simulink model "arducopter"  (R2024b)
settings: Solver=FixedStepAuto  StartTime=0.0  StopTime=simIn.param.timeEnd  FixedStep=simIn.param.dt  RelTol=1e-3
undefined symbols (not defined in the file or in its folder): DiscIntNeverNeededParam, sim, simIn
libraries: simulink x60, slident x4, vrlib x1
(part 6 of 9)

== system arducopter/Rate Controller/PID Yaw Rate/Slew Limiter ==
  note: Data Store Memory Elements: Global variables of subsystem
  note: Slew Limiter
      |
      | Calculates the slew limit modifiert Dmod for the P and D part of the controller. The calculation of Dmod is taken from SlewLimiter::modifier() in SlewLimiter.cpp.
  note: Alpha Calculation:
      | $\alpha = \frac{\mathrm{d}t}{\mathrm{d}t + 2 \pi f_{\mathrm{Cutoff}}$
  note: See AP_Math.cpp, calc_lowpass_alpha_dt()
  p_out : Inport
  sr_max : Inport  Port=2
  sr_tau : Inport  Port=3
  sr_flt_f : Inport  Port=4
  clock : Inport  Port=5
  d_out : Inport  Port=6
  ATC input time constant : Constant  Value=simIn.param.dt
  Add1 : Sum
  Calculate Alpha : Product  Inputs=*/
  Calculate Dmod : MATLAB Function  TreatAsAtomicUnit=on  SystemSampleTime=0.0025
  Compare To Zero2 : simulink/Logic and Bit Operations/Compare To Zero  relop=<=  OutDataTypeStr=boolean
  Compare To Zero3 : simulink/Logic and Bit Operations/Compare To Zero  relop=<=  OutDataTypeStr=boolean
  Compare To Zero4 : simulink/Logic and Bit Operations/Compare To Zero  relop=~=  OutDataTypeStr=boolean
  Constant1 : Constant  OutDataTypeStr=single
  Constant5 : Constant  OutDataTypeStr=single
  Data Store Memory : DataStoreMemory  DataStoreName=pos_event_stored  ReadBeforeWriteMsg=warning  WriteAfterWriteMsg=warning  WriteAfterReadMsg=warning  InitialValue=false  ShowAdditionalParam=off  OutDataTypeStr=boolean
  Data Store Memory1 : DataStoreMemory  DataStoreName=neg_event_stored  ReadBeforeWriteMsg=warning  WriteAfterWriteMsg=warning  WriteAfterReadMsg=warning  InitialValue=false  ShowAdditionalParam=off  OutDataTypeStr=boolean
  Data Store Memory10 : DataStoreMemory  DataStoreName=modifier_slew_rate  ReadBeforeWriteMsg=warning  WriteAfterWriteMsg=warning  WriteAfterReadMsg=warning  InitialValue=simIn.init.PIDY.SROut  ShowAdditionalParam=off  OutDataTypeStr=single
  Data Store Memory11 : DataStoreMemory  DataStoreName=output_slew_rate  ReadBeforeWriteMsg=warning  WriteAfterWriteMsg=warning  WriteAfterReadMsg=warning  InitialValue=simIn.init.PIDY.SROut  ShowAdditionalParam=off  OutDataTypeStr=single
  Data Store Memory2 : DataStoreMemory  DataStoreName=pos_event_idx  ReadBeforeWriteMsg=warning  WriteAfterWriteMsg=warning  WriteAfterReadMsg=warning  InitialValue=1  ShowAdditionalParam=off  OutDataTypeStr=int8
  Data Store Memory3 : DataStoreMemory  DataStoreName=neg_event_idx  ReadBeforeWriteMsg=warning  WriteAfterWriteMsg=warning  WriteAfterReadMsg=warning  InitialValue=1  ShowAdditionalParam=off  OutDataTypeStr=int8
  Data Store Memory4 : DataStoreMemory  DataStoreName=pos_event_ms  ReadBeforeWriteMsg=warning  WriteAfterWriteMsg=warning  WriteAfterReadMsg=warning  InitialValue=[0 0]  ShowAdditionalParam=off  OutDataTypeStr=uint32  Dimensions=2
  Data Store Memory5 : DataStoreMemory  DataStoreName=neg_event_ms  ReadBeforeWriteMsg=warning  WriteAfterWriteMsg=warning  WriteAfterReadMsg=warning  InitialValue=[0 0]  ShowAdditionalParam=off  OutDataTypeStr=uint32  Dimensions=2
  Data Store Memory6 : DataStoreMemory  DataStoreName=max_pos_slew_rate  ReadBeforeWriteMsg=warning  WriteAfterWriteMsg=warning  WriteAfterReadMsg=warning  ShowAdditionalParam=off  OutDataTypeStr=single
  Data Store Memory7 : DataStoreMemory  DataStoreName=max_pos_slew_event_ms  ReadBeforeWriteMsg=warning  WriteAfterWriteMsg=warning  WriteAfterReadMsg=warning  ShowAdditionalParam=off  OutDataTypeStr=uint32
  Data Store Memory8 : DataStoreMemory  DataStoreName=max_neg_slew_rate  ReadBeforeWriteMsg=warning  WriteAfterWriteMsg=warning  WriteAfterReadMsg=warning  ShowAdditionalParam=off  OutDataTypeStr=single
  Data Store Memory9 : DataStoreMemory  DataStoreName=max_neg_slew_event_ms  ReadBeforeWriteMsg=warning  WriteAfterWriteMsg=warning  WriteAfterReadMsg=warning  ShowAdditionalParam=off  OutDataTypeStr=uint32
  Data Store Read : DataStoreRead  DataStoreName=modifier_slew_rate  DataStoreElements=modifier_slew_rate  IndexOptions=Index vector (dialog)  Indices=1  OutputSizes=1
  Data Store Read1 : DataStoreRead  DataStoreName=output_slew_rate  DataStoreElements=output_slew_rate  IndexOptions=Index vector (dialog)  Indices=1  OutputSizes=1
  Data Type Conversion2 : DataTypeConversion  OutDataTypeStr=single  SaturateOnIntegerOverflow=off  RndMeth=Floor
  Divide1 : Product  Inputs=*/
  Gain1 : Gain  Gain=2*pi
  IC : InitialCondition  Value=2*simIn.init.PIDY.SROut
  Logical Operator1 : Logic  Operator=OR  AllPortsSameDT=off  OutDataTypeStr=boolean
  Lowpass Filter : MATLAB Function  TreatAsAtomicUnit=on
  Product2 : Product
  Subsystem : Subsystem
  Switch1 : Switch  Criteria=u2 > Threshold  SaturateOnIntegerOverflow=off  InputSameDT=off
  Terminator : Terminator
  Terminator1 : Terminator
  Unit Delay1 : UnitDelay  SampleTime=-1  HasFrameUpgradeWarning=on
  Dmod : Outport
  wires:
  Lowpass Filter/1(out) -> IC/1  "yawRateSrFilt"
  Unit Delay1/1 -> Lowpass Filter/3(out_last)
  Calculate Dmod/1(Dmod) -> Dmod/1  "yawRateDmod"
  sr_max/1 -> Calculate Dmod/2(sr_max)
  sr_tau/1 -> Calculate Dmod/3(sr_tau)
  Data Store Read/1 -> Terminator/1  "yawRateSrModifier"
  Data Store Read1/1 -> Terminator1/1  "yawRateSrOut"
  p_out/1 -> Subsystem/1(p_out)
  d_out/1 -> Subsystem/2(d_out)
  Subsystem/1(sr_raw) -> Lowpass Filter/1(in)  "yawRateSrRaw"
  IC/1 -> Calculate Dmod/1(slew_rate), Unit Delay1/1
  clock/1 -> Calculate Dmod/5(time)
  [cutoff_freq] -> Gain1/1
  [dt] -> Calculate Alpha/1, Add1/1
  Calculate Alpha/1 -> Switch1/3
  Gain1/1 -> Divide1/2
  Data Type Conversion2/1 -> [dt]
  ATC input time constant/1 -> Data Type Conversion2/1
  [cutoff_freq] -> Compare To Zero3/1
  Compare To Zero3/1 -> Logical Operator1/2
  Constant1/1 -> Divide1/1
  [dt] -> Compare To Zero2/1
  Logical Operator1/1 -> Switch1/2
  Compare To Zero2/1 -> Logical Operator1/1
  Add1/1 -> Calculate Alpha/2
  Divide1/1 -> Add1/2
  Product2/1 -> Switch1/1
  [dt] -> Compare To Zero4/1
  Switch1/1 -> Lowpass Filter/2(alpha)
  Compare To Zero4/1 -> Product2/1
  Constant5/1 -> Product2/2
  sr_flt_f/1 -> [cutoff_freq]
  [dt] -> Calculate Dmod/4(dt)

== system arducopter/Throttle/Throttle Calculations/Air density Calculation ==
  note: Calculation of the air density from the barometer signals.
      |
      | In order to determine the compensation gain, the air density ratio is calculated in this subsystem from the barometer measurement signals. This subsystem is only used for validation purposes.
      |
      | The calculations are based on the get_air_density_ratio() function in AP_AHRS.cpp and the _get_EAS2TAS() function (AP_Baro_atmosphere.cpp), which is called from there. The variable air_density_ratio for the air density ratio, which is used for the calculation of the compensation gain, is set in the ahrs() object.
  baroAlt : Inport
  baroAirPress : Inport  Port=2
  baroGndTemp : Inport  Port=3
  Data Store Memory : DataStoreMemory  DataStoreName=EAS2TAS  ReadBeforeWriteMsg=warning  WriteAfterWriteMsg=warning  WriteAfterReadMsg=warning  ShowAdditionalParam=off  OutDataTypeStr=single
  Data Store Memory1 : DataStoreMemory  DataStoreName=last_alt_EAS2TAS  ReadBeforeWriteMsg=warning  WriteAfterWriteMsg=warning  WriteAfterReadMsg=warning  ShowAdditionalParam=off  OutDataTypeStr=single
  Get air density ratio : MATLAB Function  TreatAsAtomicUnit=on
  Get equivalent to true airspeed EAS2TAS : MATLAB Function  TreatAsAtomicUnit=on  SystemSampleTime=simIn.param.dt
  airDensityRatio : Outport
  wires:
  Get equivalent to true airspeed EAS2TAS/1(eas2tas) -> Get air density ratio/1(eas2tas)
  Get air density ratio/1(airDensityRatio) -> airDensityRatio/1
  baroAlt/1 -> Get equivalent to true airspeed EAS2TAS/1(alt)
  baroAirPress/1 -> Get equivalent to true airspeed EAS2TAS/2(airPress)
  baroGndTemp/1 -> Get equivalent to true airspeed EAS2TAS/3(gndTemp)

== system arducopter/Throttle/Throttle Calculations/Boost and Premixing ==
  note: Consider implementing whole get_throttle_boosted() function because currently only the measured angle_boost is used and angle_boost isn't calculated in the simulation
  note: Angular boost and premixing.
  note: This function adds the angular boost to the desired throttle (if enabled) and outputs the maximum value between the desired throttle and the throttle, that results from mixing the desired throttle with the hover throttle.
      | (set_throttle_out() function in AC_AttitudeControl_Multi.cpp)
      | It is either called from the flightmode->run() function, if the flightmode does not include position control, or from the update_z_controller() function in AC_PosControl.cpp if position control is used.
  thrRPYMix : Inport
  thrIn : Inport  Port=2
  thrHover : Inport  Port=3
  angBst : Inport  Port=4
  Constant9 : Constant  Value=simIn.param.ATC.ANGLE_BOOST
  Throttle_In Handling : MATLAB Function  TreatAsAtomicUnit=on
  thrOutRaw : Outport
  thrAvgMax : Outport  Port=2
  wires:
  Constant9/1 -> Throttle_In Handling/4(angBstEna)
  Throttle_In Handling/2(thrAvgMax) -> thrAvgMax/1
  thrIn/1 -> Throttle_In Handling/1(thrTar)
  angBst/1 -> Throttle_In Handling/2(angBst)
  thrRPYMix/1 -> Throttle_In Handling/5(thrRpyMix)
  thrHover/1 -> Throttle_In Handling/3(thrHover)
  Throttle_In Handling/1(thrOut) -> thrOutRaw/1  "thrOutRaw"

== system arducopter/Throttle/Throttle Calculations/Lowpass Filter ==
  note: what init value for unit delay?
  note: Lowpass filter throttle
      | This lowpass filter for the throttle is called in AP_MotorsMulticopter::update_throttle_filter() (AP_MotorsMulticoopter.cpp), which
      | is called in AP_MotorsMulticopter::output(), which is in turn called from Copter::motors_output in motors.cpp through output_to_motors() in mode.cpp.
  thrOutRaw : Inport
  Constant2 : Constant  Value=simIn.param.dt  OutDataTypeStr=single
  Constant8 : Constant  Value=simIn.param.ATC.THR_FILT_CUTOFF  OutDataTypeStr=single
  Data Type Conversion : DataTypeConversion  OutDataTypeStr=single  SaturateOnIntegerOverflow=off  RndMeth=Floor
  Lowpass Filter with reset : MATLAB Function  TreatAsAtomicUnit=on
  Unit Delay : UnitDelay  SampleTime=-1  HasFrameUpgradeWarning=on
  Unit Delay1 : UnitDelay  InitialCondition=simIn.init.CTUN.ThrOut  SampleTime=-1  HasFrameUpgradeWarning=on
  thrOutFilt : Outport
  thrSlewRate : Outport  Port=2
  wires:
  Constant8/1 -> Lowpass Filter with reset/2(cutoff_freq)
  Constant2/1 -> Lowpass Filter with reset/3(dt)
  Unit Delay1/1 -> Lowpass Filter with reset/4(lastThr)
  thrOutRaw/1 -> Lowpass Filter with reset/1(thr_in)
  Lowpass Filter with reset/1(out) -> Unit Delay1/1, thrOutFilt/1  "thrOutFilt"
  Lowpass Filter with reset/2(slewrate) -> thrSlewRate/1, Unit Delay/1
  Unit Delay/1 -> Data Type Conversion/1
  Data Type Conversion/1 -> Lowpass Filter with reset/5(lastSlew)

== system arducopter/Throttle/Throttle Calculations/Throttle Hover ==
  note: Update throttle hover
  note: The parameters THST_HOVER_TC, THST_HOVER_MIN and THST_HOVER_MAX are defined in AP_MotorsMulticopter.h. The value 0.01 for dt is taken from the function call Copter::update_throttle_hover() in Attitude.cpp.
      | The parameters THST_HOVER and HOVER_LEARN are defined in AP_MotorsMulticopter.cpp. They are set in the initialization of the copter with the parameters MOT_THST_HOVER and MOT_THST_LEARN
      | respectively.
  note: Subsystem for updating throttle hover. Runs as a atomic unit with a sample time of 10 ms (100 Hz) since the scheduler task for updating the throttle hover value is called with this frequency (see Copter.cpp, SCHED_TASK(update_throttle_hover, 100, 90) ).
      | Simply uses the default hover value, when manual throttle is active (as the first condition) or thr_hover_learn is not activated (as the secondary condition).
  zVelAct : Inport
  zVelDes : Inport  Port=2
  thrAct : Inport  Port=3
  Constant : Constant  Value=0.01  OutDataTypeStr=single
  Constant1 : Constant  Value=simIn.param.MOT.THST_HOVER_MAX
  Constant2 : Constant  Value=simIn.param.MOT.THST_HOVER_MIN
  Constant3 : Constant  Value=simIn.param.MOT.THST_HOVER_TC
  Constant4 : Constant  Value=simIn.param.MOT.THST_HOVER
  Constant5 : Constant  Value=simIn.param.MOT.HOVER_LEARN
  Constant6 : Constant  Value=simIn.param.MODE.THR_MAN_FLG
  Data Store Memory : DataStoreMemory  DataStoreName=thrHoverAct  ReadBeforeWriteMsg=warning  WriteAfterWriteMsg=warning  WriteAfterReadMsg=warning  InitialValue=simIn.init.CTUN.ThrHov  ShowAdditionalParam=off  OutDataTypeStr=single
  Throttle Hover Calculation : MATLAB Function  TreatAsAtomicUnit=on
  thrHover : Outport
  wires:
  Throttle Hover Calculation/1(thrHover) -> thrHover/1  "thrHover"
  Constant/1 -> Throttle Hover Calculation/1(dt)
  thrAct/1 -> Throttle Hover Calculation/2(thrAct)
  Constant1/1 -> Throttle Hover Calculation/5(thstHoverMax)
  Constant2/1 -> Throttle Hover Calculation/6(thstHoverMin)
  Constant3/1 -> Throttle Hover Calculation/7(thstHoverTC)
  Constant4/1 -> Throttle Hover Calculation/8(thstHoverDefault)
  Constant5/1 -> Throttle Hover Calculation/9(hoverLearn)
  Constant6/1 -> Throttle Hover Calculation/10(thrMan)
  zVelAct/1 -> Throttle Hover Calculation/4(zVelAct)
  zVelDes/1 -> Throttle Hover Calculation/3(zVelDes)

== system arducopter/Throttle/Throttle Calculations/Throttle Limiting based on battery state ==
  note: thr_limit and thr_thst_max are set to 1.0 as initial value, since both values are set to 1.0
      | when the motors are disarmed (see get_current_limit_max_throttle()), which
      | means both quantities are always set to 1.0 at the beginning of a flight.
  note: Calculates the throttle limit that represents the maximum additional throttle on top of the hover throttle based on the ratio between actual and maximum battery current. The higher the ratio (and the higher the utilization repectively), the lower the throttle limit. The acutal current is taken as minimum for the limit.
  note: Calculates maximum lift "lift_max" based on resting battery voltage (battery voltage reduced by sag that results from internal resistance, calculated in AP_BattMonitor_Backend.cpp, update_resistance_estimate()) and sets a new lower limit for the voltage "bat_volt_min" below that no additional scaling of thrust is conducted.
  note: Calculation of quantities to limit or scale thrust output.
  batRestVoltEst : Inport
  batCurr : Inport  Port=2
  batRes : Inport  Port=3
  batVolt : Inport  Port=4
  thrHover : Inport  Port=5
  Constant11 : Constant  Value=simIn.param.LOOP_RATE
  Constant12 : Constant  Value=simIn.param.MOT.THST_EXPO
  Constant13 : Constant  Value=simIn.param.MOT.BAT_VOLT_MIN
  Constant14 : Constant  Value=simIn.param.MOT.BAT_VOLT_MAX
  Constant15 : Constant  Value=simIn.param.LOOP_RATE
  Constant16 : Constant  Value=simIn.param.MOT.BAT_CURR_MAX
  Constant17 : Constant  Value=simIn.param.MOT.BAT_CURR_TC
  Get current throttle limit : MATLAB Function  TreatAsAtomicUnit=on
  IC : InitialCondition
  Unit Delay3 : UnitDelay  InitialCondition=simIn.init.BAT.RestVoltEst/simIn.param.MOT.BAT_VOLT_MIN  SampleTime=-1  HasFrameUpgradeWarning=on
  Unit Delay4 : UnitDelay  InitialCondition=1.0  SampleTime=-1  HasFrameUpgradeWarning=on
  Update Lift Max from Battery Voltage : MATLAB Function  TreatAsAtomicUnit=on
  liftMax : Outport
  batVoltRestEstAct : Outport  Port=2
  thrThstMax : Outport  Port=3
  wires:
  Unit Delay3/1 -> Update Lift Max from Battery Voltage/1(battVoltFiltLast)
  Constant16/1 -> Get current throttle limit/2(batCurrMax)
  Constant17/1 -> Get current throttle limit/3(batCurrT)
  batVolt/1 -> Get current throttle limit/7(batVolt)
  Update Lift Max from Battery Voltage/1(battVoltFilt) -> Unit Delay3/1
  Constant14/1 -> Update Lift Max from Battery Voltage/3(battVoltMax)
  thrHover/1 -> Get current throttle limit/8(thrHover)
  Constant13/1 -> Update Lift Max from Battery Voltage/4(battVoltMin)
  Update Lift Max from Battery Voltage/3(battVoltMinAct) -> Get current throttle limit/1(batVoltMin)
  batRestVoltEst/1 -> Update Lift Max from Battery Voltage/2(battVoltRestEst)
  Update Lift Max from Battery Voltage/2(liftMax) -> liftMax/1
  batCurr/1 -> Get current throttle limit/5(batCurr)
  Constant12/1 -> Update Lift Max from Battery Voltage/5(thstCurveExpo)
  Constant15/1 -> Get current throttle limit/4(loop_rate)
  Unit Delay4/1 -> Get current throttle limit/9(thrLimitLast)
  batRes/1 -> Get current throttle limit/6(batRes)
  Get current throttle limit/2(thrLimit) -> Unit Delay4/1  "thrLimit"
  Constant11/1 -> Update Lift Max from Battery Voltage/6(loop_rate)
  Get current throttle limit/1(thrThstMax) -> IC/1
  Update Lift Max from Battery Voltage/4(battVoltRestEstAct) -> batVoltRestEstAct/1
  IC/1 -> thrThstMax/1

== system arducopter/Throttle/Throttle Calculations/Throttle-Attitude-Mixing ==
  note: This function limits the rate that thr_mix is rising with when thr_mix_des changes. It represents the function update_throttle_rpy_mix() in AC_AttitudeControl_Multi.cpp.
  note: Rate limiting of thr_mix
  note: Determination of thr_mix_des
  note: This function determines the priorization between throttle and attitude control based on the flight mode and current control demands.
      | High values favour attitude over throttle control.
      | Runs with 50 Hz.
      | ToDo: Add remaining conditions .
  thrIn : Inport
  zVelCtrlRatio : Inport  Port=2
  zVelDes : Inport  Port=3
  thrMixOut : Inport  Port=4
  thrMan : Inport  Port=5
  thrFiltIn : Inport  Port=6
  thrHover : Inport  Port=7
  Constant1 : Constant  Value=simIn.param.ATC.THR_MIX_MAX
  Constant10 : Constant  Value=1 / simIn.param.LOOP_RATE
  Constant2 : Constant  Value=simIn.param.ATC.THR_MIX_MIN
  Constant3 : Constant  Value=simIn.param.ATC.THR_MIX_MAN
  Constant4 : Constant  Value=simIn.param.ATC.THR_MIX_MAX
  Constant5 : Constant  Value=simIn.param.ATC.THR_MIX_MIN
  Data Store Memory : DataStoreMemory  DataStoreName=thrMixAct  ReadBeforeWriteMsg=warning  WriteAfterWriteMsg=warning  WriteAfterReadMsg=warning  InitialValue=simIn.init.ATC.THR_MIX  ShowAdditionalParam=off  OutDataTypeStr=single
  Update Throttle Mix : MATLAB Function  TreatAsAtomicUnit=on
  Update Throttle Mix Des : MATLAB Function  TreatAsAtomicUnit=on  SystemSampleTime=simIn.param.dt_THR_LOOP
  get_throttle_hover : Subsystem
  thrRPYMix : Outport
  wires:
  Constant1/1 -> Update Throttle Mix Des/6(thrMixMax)
  thrIn/1 -> Update Throttle Mix Des/1(thrTar)
  Update Throttle Mix Des/1(thrMixDes) -> Update Throttle Mix/1(thrMixDes)
  Constant2/1 -> Update Throttle Mix Des/5(thrMixMin)
  Constant10/1 -> Update Throttle Mix/7(dt)
  Constant3/1 -> Update Throttle Mix Des/7(thrMixMan)
  Constant5/1 -> Update Throttle Mix/2(thrMixMin)
  zVelCtrlRatio/1 -> Update Throttle Mix Des/2(zVelCtrlRatio)
  Constant4/1 -> Update Throttle Mix/3(thrMixMax)
  Update Throttle Mix/1(thrMix) -> thrRPYMix/1
  zVelDes/1 -> Update Throttle Mix Des/3(zVelDes)
  thrMan/1 -> Update Throttle Mix Des/4(thrMan)
  thrMixOut/1 -> Update Throttle Mix/4(thrOut)
  thrFiltIn/1 -> Update Throttle Mix/5(thrIn)
  thrHover/1 -> get_throttle_hover/1(in)
  get_throttle_hover/1(out) -> Update Throttle Mix/6(thrHover)

== system arducopter/Attitude Controller/input_euler_angle_roll_pitch_euler_rate_yaw()/Feedforward enabled/input shaping ==
  note: This subsystem contains all the function that are called for the input shaping of the desired attitude to calculate the target euler rates
  eulerAngleTar : Inport
  eulerInputDes : Inport  Port=2
  eulerRateTarIn : Inport  Port=3
  eulerAccelMax : Inport  Port=4
  Mux : Mux  Inputs=3
  Selector1 : Selector  InputPortWidth=3  IndexOptions=Index vector (dialog)  Indices=[1]  OutputSizes=1
  Selector2 : Selector  InputPortWidth=3  IndexOptions=Index vector (dialog)  Indices=[1]  OutputSizes=1
  Selector3 : Selector  InputPortWidth=3  IndexOptions=Index vector (dialog)  Indices=[3]  OutputSizes=1
  Selector4 : Selector  InputPortWidth=3  IndexOptions=Index vector (dialog)  Indices=[2]  OutputSizes=1
  Selector5 : Selector  InputPortWidth=3  IndexOptions=Index vector (dialog)  Indices=[2]  OutputSizes=1
  Selector6 : Selector  InputPortWidth=3  IndexOptions=Index vector (dialog)  Indices=[3]  OutputSizes=1
  Selector7 : Selector  InputPortWidth=3  IndexOptions=Index vector (dialog)  Indices=[1]  OutputSizes=1
  Selector8 : Selector  InputPortWidth=3  IndexOptions=Index vector (dialog)  Indices=[2]  OutputSizes=1
  Selector9 : Selector  InputPortWidth=3  IndexOptions=Index vector (dialog)  Indices=[3]  OutputSizes=1
  Subtract : Sum  Inputs=-+
  input shaping pitch angle : Subsystem
  input shaping roll angle : Subsystem
  input shaping yaw rate : Subsystem
  eulerRateTar : Outport
  wires:
  eulerAngleTar/1 -> Subtract/1
  eulerInputDes/1 -> Selector6/1, Subtract/2
  Subtract/1 -> Selector4/1, Selector1/1
  eulerAccelMax/1 -> Selector2/1, Selector3/1, Selector5/1
  Selector1/1 -> input shaping roll angle/1(rollAngleErr)
  Selector2/1 -> input shaping roll angle/3(rollAccelMax)
  Selector3/1 -> input shaping yaw rate/3(eulerAccelMax)
  Selector6/1 -> input shaping yaw rate/1(yawRateDes)
  eulerRateTarIn/1 -> Selector8/1, Selector9/1, Selector7/1
  Selector7/1 -> input shaping roll angle/2(rollRateTarIn)
  Selector4/1 -> input shaping pitch angle/1(pitchAngleErr)
  Selector5/1 -> input shaping pitch angle/3(pitchAccelMax)
  Selector8/1 -> input shaping pitch angle/2(pitchRateTarIn)
  Selector9/1 -> input shaping yaw rate/2(yawRateTar)
  Mux/1 -> eulerRateTar/1
  input shaping roll angle/1(eulerRollRateTar) -> Mux/1
  input shaping pitch angle/1(eulerPitchRateTar) -> Mux/2
  input shaping yaw rate/1(eulerYawRateTar) -> Mux/3

== system arducopter/Attitude Controller/input_euler_angle_roll_pitch_euler_rate_yaw()/Update attitudeTarget/Rotate target attitude ==
  attitudeTarget : Inport
  angVelTar : Inport  Port=2
  Constant : Constant  Value=simIn.param.dt
  MATLAB Function1 : MATLAB Function  TreatAsAtomicUnit=on
  MATLAB Function5 : MATLAB Function  TreatAsAtomicUnit=on
  Product : Product
  attitudeTargetRot : Outport
  wires:
  Product/1 -> MATLAB Function5/1(vec)
  angVelTar/1 -> Product/1
  Constant/1 -> Product/2
  MATLAB Function5/1(q) -> MATLAB Function1/2(q2)  "attitudeTargetUpdate"
  attitudeTarget/1 -> MATLAB Function1/1(q1)
  MATLAB Function1/1(qRes) -> attitudeTargetRot/1  "attitudeTargetRot"

== system arducopter/Attitude Controller/input_euler_angle_roll_pitch_euler_rate_yaw()/thrust_heading_rotation_angles()/Yaw error limitation ==
  note: schauen ob Beschreibungen zur Funktion noch passen
  note: Output adapted attitudeTarget and attitudeError if yaw limiting condition is met. Otherwise output old values.
  note: First limiting condition: if(!is_zero(get_rate_yaw_pid().kP()))
  note: Limiting of the yaw error based on the maximum allowed yaw acceleration.
      | attitudeError and attitudeTarget are updated to include the applied limits.
  attitudeErrorIn : Inport
  attitudeTargetIn : Inport  Port=2
  thrustVecCorrection : Inport  Port=3
  attitudeBody : Inport  Port=4
  Constant5 : Constant  Value=simIn.param.PIDY.P
  IsNonZero1 : simulink/Logic and Bit Operations/Compare To Zero  relop=~=  OutDataTypeStr=boolean
  "Second limiting condition " : Subsystem
  Switch : Switch  Criteria=u2 > Threshold  SaturateOnIntegerOverflow=off  InputSameDT=off
  Switch1 : Switch  Criteria=u2 > Threshold  SaturateOnIntegerOverflow=off  InputSameDT=off
  attitudeTarget : Outport
  attitudeError : Outport  Port=2
  wires:
  attitudeErrorIn/1 -> [attitudeError]
  [attitudeError] -> "Second limiting condition "/1(attitudeErrorIn)
  thrustVecCorrection/1 -> "Second limiting condition "/3(thrustVecCorrection)
  attitudeBody/1 -> "Second limiting condition "/4(attitudeBody)
  [attitudeTarget] -> Switch/3
  [attitudeError] -> Switch1/3
  Switch/1 -> attitudeTarget/1
  Switch1/1 -> attitudeError/1
  Constant5/1 -> IsNonZero1/1
  IsNonZero1/1 -> Switch1/2, Switch/2, "Second limiting condition "/Enable
  attitudeTargetIn/1 -> [attitudeTarget]
  [attitudeTarget] -> "Second limiting condition "/2(attitudeTargetIn)
  "Second limiting condition "/1(attitudeTarget) -> Switch/1
  "Second limiting condition "/2(attitudeError) -> Switch1/1

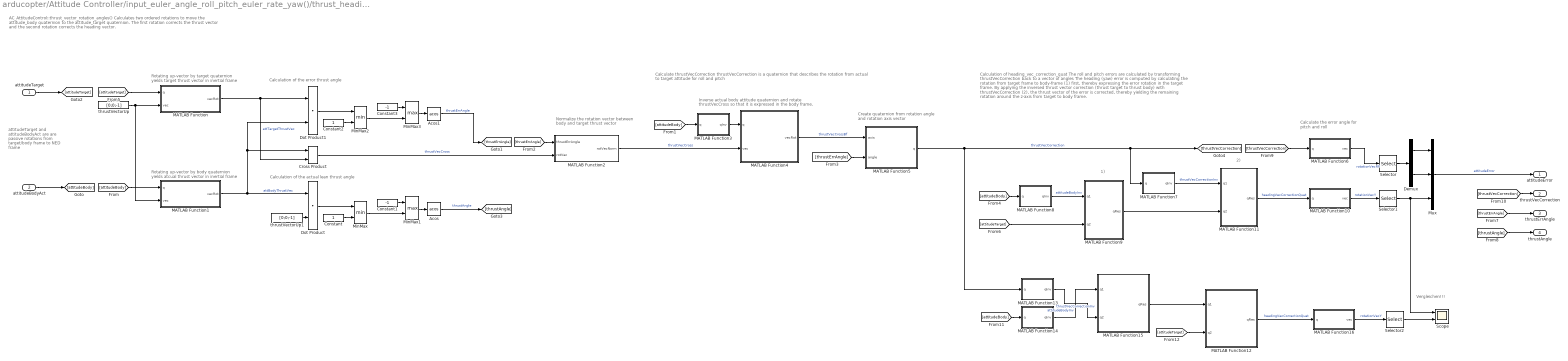
== system arducopter/Attitude Controller/input_euler_angle_roll_pitch_euler_rate_yaw()/thrust_heading_rotation_angles()/thrust_vector_rotation_angles() ==
  note: Vergleichen!!!
  note: 1)
  note: attitudeTarget and
      | attitudeBodyAct are are passive rotations from target/body frame to NED frame
  note: Calculation of heading_vec_correction_quat
      | The roll and pitch errors are calculated by transforming thrustVecCorrection back to a vector of angles
      | The heading (yaw) error is computed by calculating the rotation from target frame to body-frame (1) first, thereby expressing the error rotation in the target frame. By applying the inversed thrust vector correction (thrust target to thrust body) with thrustVecCorrection (2), the thrust vector of the error is corrected, thereby yielding the remaining rotation around the z-axis from target to body frame.
  note: Create quaternion from rotation angle and rotation axis vector
  note: Inverse actual body attitude quaternion and rotate thrustVecCross so that it is expressed in the body frame.
  note: Calculate the error angle for pitch and roll
  note: Calculate thrustVecCorrection
      | thrustVecCorrection is a quaternion that describes the rotation from actual to target attitude for roll and pitch
  note: Normalize the rotation vector between body and target thrust vector
  note: Calculation of the actual lean thrust angle
  note: Rotating up-vector by target quaternion
      | yields target thrust vector in inertial frame
  note: AC_AttitudeControl::thrust_vector_rotation_angles()
      | Calculates two ordered rotations to move the attitude_body quaternion to the attitude_target quaternion. The first rotation corrects the thrust vector and the second rotation corrects the heading vector.
  note: Rotating up-vector by body quaternion
      | yields atcual thrust vector in inertial frame
  note: Calculation of the error thrust angle
  note: 2)
  attitudeTarget : Inport
  attitudeBodyAct : Inport  Port=2
  Acos : Trigonometry  Operator=acos
  Acos1 : Trigonometry  Operator=acos
  Constant : Constant  OutDataTypeStr=single
  Constant1 : Constant  Value=-1  OutDataTypeStr=single
  Constant2 : Constant  OutDataTypeStr=single
  Constant3 : Constant  Value=-1  OutDataTypeStr=single
  Cross Product : vrlib/Utilities/Cross Product
  Demux : Demux  Outputs=2
  Dot Product : DotProduct  OutDataTypeStr=Inherit: Inherit via internal rule
  Dot Product1 : DotProduct  OutDataTypeStr=Inherit: Inherit via internal rule
  MATLAB Function : MATLAB Function  TreatAsAtomicUnit=on
  MATLAB Function1 : MATLAB Function  TreatAsAtomicUnit=on
  MATLAB Function10 : MATLAB Function  TreatAsAtomicUnit=on
  MATLAB Function11 : MATLAB Function  TreatAsAtomicUnit=on
  MATLAB Function12 : MATLAB Function  TreatAsAtomicUnit=on
  MATLAB Function13 : MATLAB Function  TreatAsAtomicUnit=on
  MATLAB Function14 : MATLAB Function  TreatAsAtomicUnit=on
  MATLAB Function15 : MATLAB Function  TreatAsAtomicUnit=on
  MATLAB Function16 : MATLAB Function  TreatAsAtomicUnit=on
  MATLAB Function2 : MATLAB Function  TreatAsAtomicUnit=on
  MATLAB Function3 : MATLAB Function  TreatAsAtomicUnit=on
  MATLAB Function4 : MATLAB Function  TreatAsAtomicUnit=on
  MATLAB Function5 : MATLAB Function  TreatAsAtomicUnit=on
  MATLAB Function6 : MATLAB Function  TreatAsAtomicUnit=on
  MATLAB Function7 : MATLAB Function  TreatAsAtomicUnit=on
  MATLAB Function8 : MATLAB Function  TreatAsAtomicUnit=on
  MATLAB Function9 : MATLAB Function  TreatAsAtomicUnit=on
  MinMax : MinMax  Inputs=2
  MinMax1 : MinMax  Function=max  Inputs=2
  MinMax2 : MinMax  Inputs=2
  MinMax3 : MinMax  Function=max  Inputs=2
  Mux : Mux  Inputs=3
  Scope : Scope  NumInputPorts=2
  Selector : Selector  InputPortWidth=3  IndexOptions=Index vector (dialog)  Indices=[1 2]  OutputSizes=1
  Selector1 : Selector  InputPortWidth=3  IndexOptions=Index vector (dialog)  Indices=[3]  OutputSizes=1
  Selector2 : Selector  InputPortWidth=3  IndexOptions=Index vector (dialog)  Indices=[3]  OutputSizes=1
  thrustVectorUp : Constant  Value=[0;0;-1]  OutDataTypeStr=single
  thrustVectorUp1 : Constant  Value=[0;0;-1]  OutDataTypeStr=single
  attitudeError : Outport
  thrustVecCorrection : Outport  Port=2
  thrustErrAngle : Outport  Port=3
  thrustAngle : Outport  Port=4
  wires:
  attitudeTarget/1 -> [attitudeTarget]
  thrustVectorUp/1 -> MATLAB Function1/2(vec), MATLAB Function/2(vec)
  [attitudeBody] -> MATLAB Function1/1(q)
  MATLAB Function/1(vecRot) -> Cross Product/2, Dot Product1/1  "attTargetThrustVec"
  MATLAB Function1/1(vecRot) -> Dot Product/1, Cross Product/1, Dot Product1/2  "attBodyThrustVec"
  Dot Product/1 -> MinMax/1
  MinMax/1 -> MinMax1/2
  Constant/1 -> MinMax/2
  Constant1/1 -> MinMax1/1
  MinMax1/1 -> Acos/1
  thrustVectorUp1/1 -> Dot Product/2
  Acos/1 -> [thrustAngle]  "thrustAngle"
  Constant2/1 -> MinMax2/2
  Dot Product1/1 -> MinMax2/1
  Constant3/1 -> MinMax3/1
  MinMax3/1 -> Acos1/1
  MinMax2/1 -> MinMax3/2
  Cross Product/1 -> MATLAB Function2/2(rotVec)  "thrustVecCross"
  Acos1/1 -> [thrustErrAngle]  "thrustErrAngle"
  attitudeBodyAct/1 -> [attitudeBody]
  [attitudeBody] -> MATLAB Function3/1(q)
  MATLAB Function2/1(rotVecNorm) -> MATLAB Function4/2(vec)  "thrustVecCross"
  MATLAB Function3/1(qInv) -> MATLAB Function4/1(q)
  [thrustErrAngle] -> MATLAB Function2/1(thrustErrAngle)
  MATLAB Function4/1(vecRot) -> MATLAB Function5/1(axis)  "thrustVecCrossBf"
  [thrustErrAngle] -> MATLAB Function5/2(angle)
  [attitudeBody] -> MATLAB Function8/1(q)
  [attitudeTarget] -> MATLAB Function/1(q)
  MATLAB Function7/1(qInv) -> MATLAB Function11/1(q1)  "thrustVecCorrectionInv"
  MATLAB Function8/1(qInv) -> MATLAB Function9/1(q1)  "attitudeBodyInv"
  [attitudeTarget] -> MATLAB Function9/2(q2)
  MATLAB Function11/1(qRes) -> MATLAB Function10/1(q)  "headingVecCorrectionQuat"
  MATLAB Function10/1(vec) -> Selector1/1  "rotationVecY"
  MATLAB Function6/1(vec) -> Selector/1  "rotationVecRP"
  Demux/1 -> Mux/1
  Demux/2 -> Mux/2
  Selector/1 -> Demux/1
  Selector1/1 -> Scope/1, Mux/3
  Mux/1 -> attitudeError/1  "attitudeError"
  [thrustErrAngle] -> thrustErrAngle/1
  [thrustAngle] -> thrustAngle/1
  [thrustVecCorrection] -> MATLAB Function6/1(q)
  [thrustVecCorrection] -> thrustVecCorrection/1
  [attitudeTarget] -> MATLAB Function12/2(q2)
  MATLAB Function15/1(qRes) -> MATLAB Function12/1(q1)
  MATLAB Function14/1(qInv) -> MATLAB Function15/1(q1)  "attitudeBodyInv"
  MATLAB Function13/1(qInv) -> MATLAB Function15/2(q2)  "thrustVecCorrectionInv"
  [attitudeBody] -> MATLAB Function14/1(q)
  MATLAB Function5/1(q) -> MATLAB Function13/1(q), [thrustVecCorrection], MATLAB Function7/1(q)  "thrustVecCorrection"
  MATLAB Function9/1(qRes) -> MATLAB Function11/2(q2)
  MATLAB Function12/1(qRes) -> MATLAB Function16/1(q)  "headingVecCorrectionQuat"
  MATLAB Function16/1(vec) -> Selector2/1  "rotationVecY"
  Selector2/1 -> Scope/2

== system arducopter/Attitude Controller/input_euler_angle_roll_pitch_euler_rate_yaw()/update_ang_vel_target_from_att_error()/Calc angular velocity target pitch ==
  note: Use square root controller if maximum angular acceleration is not zero
  attitudeErrorPitch : Inport
  anglePScale : Inport  Port=2
  Constant1 : Constant  Value=simIn.param.ATC.ACCEL_P_MAX
  Constant2 : Constant  Value=simIn.param.ATC.ACCEL_RP_CONTROLLER_MAX_RADSS
  Constant3 : Constant  Value=simIn.param.ATC.ACCEL_P_MAX
  Constant4 : Constant  Value=simIn.param.ATC.ACCEL_RP_CONTROLLER_MIN_RADSS
  Constant6 : Constant  Value=simIn.param.dt  VectorParams1D=off
  Constant7 : Constant  Value=simIn.param.ATC.ANG_PIT_P
  Constant8 : Constant  Value=simIn.param.ATC.ANG_PIT_P
  Gain : Gain  Gain=0.5
  Product : Product
  Product1 : Product
  Saturation Dynamic : simulink/Discontinuities/Saturation Dynamic  OutMin=[]  OutMax=[]  OutDataTypeStr=Inherit: Same as second input  OutDataType=fixdt(1, 16)  OutScaling=2^-10  DoSatur=off
  Square Root Controller : MATLAB Function  TreatAsAtomicUnit=on
  Switch : Switch  Criteria=u2 > Threshold  SaturateOnIntegerOverflow=off  InputSameDT=off
  cdeg/ss to rad/ss1 : Gain  Gain=0.01*pi/180
  angVelPitch : Outport
  wires:
  Constant4/1 -> Saturation Dynamic/3
  Constant2/1 -> Saturation Dynamic/1
  Gain/1 -> Saturation Dynamic/2
  Constant1/1 -> Gain/1
  Saturation Dynamic/1 -> Square Root Controller/3(second_ord_lim)
  attitudeErrorPitch/1 -> Product/2, Square Root Controller/1(err)
  Product/1 -> Switch/3
  Constant6/1 -> Square Root Controller/4(dt)
  Square Root Controller/1(correction_rate) -> Switch/1
  Switch/1 -> angVelPitch/1
  Constant3/1 -> cdeg/ss to rad/ss1/1
  Constant7/1 -> Product/1
  cdeg/ss to rad/ss1/1 -> Switch/2
  Product1/1 -> Square Root Controller/2(p)
  Constant8/1 -> Product1/2
  anglePScale/1 -> Product1/1

== system arducopter/Attitude Controller/input_euler_angle_roll_pitch_euler_rate_yaw()/update_ang_vel_target_from_att_error()/Calc angular velocity target roll ==
  note: Use square root controller if maximum angular acceleration is not zero
  attitudeErrorRoll : Inport
  anglePScale : Inport  Port=2
  Constant1 : Constant  Value=simIn.param.ATC.ACCEL_R_MAX
  Constant2 : Constant  Value=simIn.param.ATC.ACCEL_RP_CONTROLLER_MAX_RADSS
  Constant3 : Constant  Value=simIn.param.ATC.ACCEL_R_MAX
  Constant4 : Constant  Value=simIn.param.ATC.ACCEL_RP_CONTROLLER_MIN_RADSS
  Constant6 : Constant  Value=simIn.param.dt  VectorParams1D=off
  Constant7 : Constant  Value=simIn.param.ATC.ANG_RLL_P
  Constant8 : Constant  Value=simIn.param.ATC.ANG_RLL_P
  Gain : Gain  Gain=0.5
  Product : Product
  Product1 : Product
  Saturation Dynamic : simulink/Discontinuities/Saturation Dynamic  OutMin=[]  OutMax=[]  OutDataTypeStr=Inherit: Same as second input  OutDataType=fixdt(1, 16)  OutScaling=2^-10  DoSatur=off
  Square Root Controller : MATLAB Function  TreatAsAtomicUnit=on
  Switch : Switch  Criteria=u2 > Threshold  SaturateOnIntegerOverflow=off  InputSameDT=off
  cdeg/ss to rad/ss1 : Gain  Gain=0.01*pi/180
  angVelRoll : Outport
  wires:
  cdeg/ss to rad/ss1/1 -> Switch/2
  Constant7/1 -> Product/1
  Constant3/1 -> cdeg/ss to rad/ss1/1
  Switch/1 -> angVelRoll/1
  Square Root Controller/1(correction_rate) -> Switch/1
  Constant6/1 -> Square Root Controller/4(dt)
  Product/1 -> Switch/3
  attitudeErrorRoll/1 -> Square Root Controller/1(err), Product/2
  Saturation Dynamic/1 -> Square Root Controller/3(second_ord_lim)
  Constant1/1 -> Gain/1
  Gain/1 -> Saturation Dynamic/2
  Constant2/1 -> Saturation Dynamic/1
  Constant4/1 -> Saturation Dynamic/3
  anglePScale/1 -> Product1/1
  Constant8/1 -> Product1/2
  Product1/1 -> Square Root Controller/2(p)

== system arducopter/Attitude Controller/input_euler_angle_roll_pitch_euler_rate_yaw()/update_ang_vel_target_from_att_error()/Calc angular velocity target yaw ==
  note: Use square root controller if maximum angular acceleration is not zero
  attitudeErrorYaw : Inport
  Constant1 : Constant  Value=simIn.param.ATC.ACCEL_Y_MAX
  Constant2 : Constant  Value=simIn.param.ATC.ACCEL_Y_CONTROLLER_MAX_RADSS
  Constant3 : Constant  Value=simIn.param.ATC.ACCEL_Y_MAX
  Constant4 : Constant  Value=simIn.param.ATC.ACCEL_Y_CONTROLLER_MIN_RADSS
  Constant6 : Constant  Value=simIn.param.dt  VectorParams1D=off
  Constant7 : Constant  Value=simIn.param.ATC.ANG_YAW_P
  Constant8 : Constant  Value=simIn.param.ATC.ANG_YAW_P
  Gain : Gain  Gain=0.5
  Product : Product
  Saturation Dynamic : simulink/Discontinuities/Saturation Dynamic  OutMin=[]  OutMax=[]  OutDataTypeStr=Inherit: Same as second input  OutDataType=fixdt(1, 16)  OutScaling=2^-10  DoSatur=off
  Square Root Controller : MATLAB Function  TreatAsAtomicUnit=on
  Switch : Switch  Criteria=u2 > Threshold  SaturateOnIntegerOverflow=off  InputSameDT=off
  cdeg/ss to rad/ss1 : Gain  Gain=0.01*pi/180
  angVelYaw : Outport
  wires:
  cdeg/ss to rad/ss1/1 -> Switch/2
  Constant7/1 -> Product/1
  Constant3/1 -> cdeg/ss to rad/ss1/1
  Constant8/1 -> Square Root Controller/2(p)
  Switch/1 -> angVelYaw/1
  Square Root Controller/1(correction_rate) -> Switch/1
  Constant6/1 -> Square Root Controller/4(dt)
  Product/1 -> Switch/3
  attitudeErrorYaw/1 -> Square Root Controller/1(err), Product/2
  Saturation Dynamic/1 -> Square Root Controller/3(second_ord_lim)
  Constant1/1 -> Gain/1
  Gain/1 -> Saturation Dynamic/2
  Constant2/1 -> Saturation Dynamic/1
  Constant4/1 -> Saturation Dynamic/3

== system arducopter/Position Controller/P Position z/Set vertical speed & acceleration limit/Inverse Square Root Controller ==
  inv_sqrt_controller : TriggerPort  TriggerType=function-call  IsSimulinkFunction=on  FunctionName=inv_sqrt_controller  FunctionVisibility=scoped  VariantControl=(inherit)
  Inverse Sqrt Controller : MATLAB Function  TreatAsAtomicUnit=on
  output : ArgIn  DisableCoverage=on  OutDataTypeStr=single  ArgumentName=output
  p : ArgIn  DisableCoverage=on  Port=2  OutDataTypeStr=single  ArgumentName=p
  D_max : ArgIn  DisableCoverage=on  Port=3  OutDataTypeStr=single  ArgumentName=D_max
  err_lim : ArgOut  DisableCoverage=on  OutDataTypeStr=single  ArgumentName=err_lim
  wires:
  Inverse Sqrt Controller/1(errLim) -> err_lim/1
  output/1 -> Inverse Sqrt Controller/1(output)
  p/1 -> Inverse Sqrt Controller/2(p)
  D_max/1 -> Inverse Sqrt Controller/3(Dmax)

== system arducopter/Position Controller/PID Acceleration z/Slew Limiter/Subsystem ==
  note: p_out + d_out * _slew_limit_scale fehlt anscheinend
  p_out : Inport
  d_out : Inport  Port=2
  ATC sample time : Constant  Value=simIn.param.dt
  Add : Sum
  Divide : Product  Inputs=*/  OutDataTypeStr=single
  Subtract : Sum  Inputs=+-
  Unit Delay : UnitDelay  InitialCondition=simIn.init.PIDR.P + simIn.init.PIDR.D  SampleTime=-1  HasFrameUpgradeWarning=on
  sr_raw : Outport
  wires:
  ATC sample time/1 -> Divide/2
  Add/1 -> Unit Delay/1, Subtract/1
  Divide/1 -> sr_raw/1
  p_out/1 -> Add/1
  Unit Delay/1 -> Subtract/2
  Subtract/1 -> Divide/1
  d_out/1 -> Add/2

== system arducopter/Position Controller/set_pos_target_z_from_climb_rate()/input_vel_accel_z/calc accMin ==
  accMax : Inport
  Constant : Constant  Value=750  OutDataTypeStr=single
  Constant1 : Constant  Value=0  OutDataTypeStr=single
  Gain : Gain  Gain=-1
  Saturation Dynamic : simulink/Discontinuities/Saturation Dynamic  OutMin=[]  OutMax=[]  OutDataTypeStr=Inherit: Same as second input  OutDataType=fixdt(1, 16)  OutScaling=2^-10  DoSatur=off
  accMin : Outport
  wires:
  accMax/1 -> Saturation Dynamic/2
  Saturation Dynamic/1 -> Gain/1
  Gain/1 -> accMin/1
  Constant/1 -> Saturation Dynamic/1
  Constant1/1 -> Saturation Dynamic/3

== system arducopter/Position Controller/set_pos_target_z_from_climb_rate()/input_vel_accel_z/shape_vel_accel ==
  note: 1)
  note: shape_vel_accel()
      | Calculates the desired acceleration as a path from the current position, velocity and acceleration to an input velocity, considering the max velocity, acceleration and jerk.
      | Calculate KPa as time constant that defines the error decay in the kinematic path as the system approaches constant acceleration
      | Calculate the preliminary desired acceleration with the square root controller
      | Limit desired acceleration based on max. acceleration and jerk
  note: 3)
  note: 2)
  vel : Inport
  acc : Inport  Port=2
  velDes : Inport  Port=3
  accDes : Inport  Port=4
  accMin : Inport  Port=5
  accMax : Inport  Port=6
  jerkMax : Inport  Port=7
  dt : Inport  Port=8
  limitTotalAccel : Inport  Port=9
  MATLAB Function : MATLAB Function  TreatAsAtomicUnit=on
  Square Root Controller : MATLAB Function  TreatAsAtomicUnit=on
  calc_KPa : MATLAB Function  TreatAsAtomicUnit=on
  accDesShaped : Outport
  wires:
  vel/1 -> calc_KPa/1(velIn)
  acc/1 -> MATLAB Function/4(accIn)
  velDes/1 -> calc_KPa/2(vel)
  accMin/1 -> [accMin]
  accMax/1 -> [accMax]
  jerkMax/1 -> [jerkMax]
  dt/1 -> [dt]
  limitTotalAccel/1 -> MATLAB Function/8(limitTotalAccel)
  calc_KPa/2(KPa) -> Square Root Controller/2(p)
  Square Root Controller/1(correction_rate) -> MATLAB Function/1(accTar)
  MATLAB Function/1(accShaped) -> accDesShaped/1
  accDes/1 -> MATLAB Function/5(acc)
  calc_KPa/1(velErr) -> Square Root Controller/1(err)
  [dt] -> Square Root Controller/4(dt)
  [jerkMax] -> Square Root Controller/3(second_ord_lim)
  [jerkMax] -> calc_KPa/5(jerkMax)
  [dt] -> MATLAB Function/7(dt)
  [jerkMax] -> MATLAB Function/6(jerkMax)
  [accMin] -> calc_KPa/3(accMin)
  [accMax] -> calc_KPa/4(accMax)
  [accMin] -> MATLAB Function/2(accMin)
  [accMax] -> MATLAB Function/3(accMax)

== system arducopter/Position Controller/set_pos_target_z_from_climb_rate()/input_vel_accel_z/update_pos_vel_accel ==
  note: update_pos_vel_accel()
      | Single axis projection of position and velocity forwards in time based on
      | a time step of dt and acceleration off acc.
  posTarIn : Inport
  velDesIn : Inport  Port=2
  accDesIn : Inport  Port=3
  limitVectorZ : Inport  Port=4
  posErr : Inport  Port=5
  velErr : Inport  Port=6
  Constant : Constant  Value=simIn.param.dt
  MATLAB Function : MATLAB Function  TreatAsAtomicUnit=on
  posTar : Outport
  velDes : Outport  Port=2
  wires:
  posTarIn/1 -> MATLAB Function/1(posIn)
  velDesIn/1 -> MATLAB Function/2(velIn)
  accDesIn/1 -> MATLAB Function/3(accIn)
  Constant/1 -> MATLAB Function/4(dt)
  MATLAB Function/1(pos) -> posTar/1
  limitVectorZ/1 -> MATLAB Function/5(limit)
  MATLAB Function/2(vel) -> velDes/1
  posErr/1 -> MATLAB Function/6(posErr)
  velErr/1 -> MATLAB Function/7(velErr)

== system arducopter/Rate Controller/PID Pitch Rate/Slew Limiter/Subsystem ==
  p_out : Inport
  d_out : Inport  Port=2
  ATC sample time : Constant  Value=simIn.param.dt
  Add : Sum
  Divide : Product  Inputs=*/  OutDataTypeStr=single
  Subtract : Sum  Inputs=+-
  Unit Delay : UnitDelay  InitialCondition=simIn.init.PIDP.P + simIn.init.PIDP.D  SampleTime=-1  HasFrameUpgradeWarning=on
  sr_raw : Outport
  wires:
  ATC sample time/1 -> Divide/2
  Add/1 -> Unit Delay/1, Subtract/1
  Divide/1 -> sr_raw/1
  p_out/1 -> Add/1
  Unit Delay/1 -> Subtract/2
  Subtract/1 -> Divide/1
  d_out/1 -> Add/2

== system arducopter/Rate Controller/PID Roll Rate/Slew Limiter/Subsystem ==
  p_out : Inport
  d_out : Inport  Port=2
  ATC sample time : Constant  Value=simIn.param.dt
  Add : Sum
  Divide : Product  Inputs=*/  OutDataTypeStr=single
  Subtract : Sum  Inputs=+-
  Unit Delay : UnitDelay  InitialCondition=simIn.init.PIDR.P + simIn.init.PIDR.D  SampleTime=-1  HasFrameUpgradeWarning=on
  sr_raw : Outport
  wires:
  ATC sample time/1 -> Divide/2
  Add/1 -> Unit Delay/1, Subtract/1
  Divide/1 -> sr_raw/1
  p_out/1 -> Add/1
  Unit Delay/1 -> Subtract/2
  Subtract/1 -> Divide/1
  d_out/1 -> Add/2

== system arducopter/Rate Controller/PID Yaw Rate/Slew Limiter/Subsystem ==
  p_out : Inport
  d_out : Inport  Port=2
  ATC sample time : Constant  Value=simIn.param.dt
  Add : Sum
  Divide : Product  Inputs=*/  OutDataTypeStr=single
  Subtract : Sum  Inputs=+-
  Unit Delay : UnitDelay  InitialCondition=simIn.init.PIDY.P + simIn.init.PIDY.D  SampleTime=-1  HasFrameUpgradeWarning=on
  sr_raw : Outport
  wires:
  ATC sample time/1 -> Divide/2
  Add/1 -> Unit Delay/1, Subtract/1
  Divide/1 -> sr_raw/1
  p_out/1 -> Add/1
  Unit Delay/1 -> Subtract/2
  Subtract/1 -> Divide/1
  d_out/1 -> Add/2

== system arducopter/Throttle/Throttle Calculations/Throttle-Attitude-Mixing/get_throttle_hover ==
  note: get_throttle_hover()
  note: Constraining of throttle hover as executed in get_throttle_hover() (AP_MotorsMulticopter.h)
  in : Inport
  Constant : Constant  Value=simIn.param.MOT.THST_HOVER_MIN
  Constant1 : Constant  Value=simIn.param.MOT.THST_HOVER_MAX
  MATLAB Function : MATLAB Function  TreatAsAtomicUnit=on
  out : Outport
  wires:
  in/1 -> MATLAB Function/1(thrHover)
  MATLAB Function/1(thrHoverLim) -> out/1
  Constant/1 -> MATLAB Function/2(thrHoverMin)
  Constant1/1 -> MATLAB Function/3(thrHoverMax)

== system arducopter/Attitude Controller/input_euler_angle_roll_pitch_euler_rate_yaw()/Feedforward enabled/input shaping/input shaping pitch angle ==
  note: AC_AttitudeControl::input_shaping_angle(float error_angle, float input_tc, float accel_max, float target_ang_vel, float desired_ang_vel, float max_ang_vel, float dt)
      | Calculation of velocity correction from an angle error. The angular velocity has acceleration and deceleration limits including basic jerk limiting using _input_tc.
      |
      | Function is called from input_shaping_angle(float error_angle, float smoothing_gain, float accel_max, float target_ang_vel, float dt) as input_shaping_angle(error_angle, smoothing_gain, accel_max, target_ang_vel, 0.0f, 0.0f, dt), so desired_ang_vel = 0 and max_ang_vel = 0
  pitchAngleErr : Inport
  pitchRateTarIn : Inport  Port=2
  pitchAccelMax : Inport  Port=3
  Constant : Constant  Value=simIn.param.dt  VectorParams1D=off
  Constant1 : Constant  Value=simIn.param.ATC.INPUT_TC  VectorParams1D=off
  Constant2 : Constant  Value=simIn.param.dt  VectorParams1D=off
  Constant3 : Constant  Value=0  VectorParams1D=off
  Data Type Conversion : DataTypeConversion  OutDataTypeStr=single  SaturateOnIntegerOverflow=off  RndMeth=Floor
  Data Type Conversion1 : DataTypeConversion  OutDataTypeStr=single  SaturateOnIntegerOverflow=off  RndMeth=Floor
  MATLAB Function : MATLAB Function  TreatAsAtomicUnit=on
  MATLAB Function1 : MATLAB Function  TreatAsAtomicUnit=on
  Square Root Controller : MATLAB Function  TreatAsAtomicUnit=on
  Square Root Controller1 : Subsystem  TreatAsAtomicUnit=on
  calc p from input_tc : Subsystem
  eulerPitchRateTar : Outport
  wires:
  MATLAB Function1/1(eulerRateTar) -> eulerPitchRateTar/1
  [accelMax] -> Square Root Controller/3(second_ord_lim)
  Square Root Controller/1(correction_rate) -> MATLAB Function1/1(desiredAngVel)
  calc p from input_tc/1(p) -> Square Root Controller/2(p)
  Constant1/1 -> calc p from input_tc/1(input_tc)
  Constant/1 -> Data Type Conversion/1
  pitchAccelMax/1 -> [accelMax]
  MATLAB Function/1(radLim) -> Square Root Controller/1(err)
  pitchAngleErr/1 -> MATLAB Function/1(radIn)
  pitchRateTarIn/1 -> MATLAB Function1/2(targetAngVel)
  Data Type Conversion/1 -> Square Root Controller/4(dt)
  Data Type Conversion1/1 -> MATLAB Function1/4(dt)
  Constant2/1 -> Data Type Conversion1/1
  Constant3/1 -> MATLAB Function1/5(input_tc)
  [accelMax] -> MATLAB Function1/3(accelMax)

== system arducopter/Attitude Controller/input_euler_angle_roll_pitch_euler_rate_yaw()/Feedforward enabled/input shaping/input shaping roll angle ==
  note: AC_AttitudeControl::input_shaping_angle(float error_angle, float input_tc, float accel_max, float target_ang_vel, float desired_ang_vel, float max_ang_vel, float dt)
      | Calculation of velocity correction from an angle error. The angular velocity has acceleration and deceleration limits including basic jerk limiting using _input_tc.
      |
      | Function is called from input_shaping_angle(float error_angle, float smoothing_gain, float accel_max, float target_ang_vel, float dt) as input_shaping_angle(error_angle, smoothing_gain, accel_max, target_ang_vel, 0.0f, 0.0f, dt), so desired_ang_vel = 0 and max_ang_vel = 0
  rollAngleErr : Inport
  rollRateTarIn : Inport  Port=2
  rollAccelMax : Inport  Port=3
  Constant : Constant  Value=simIn.param.dt  VectorParams1D=off
  Constant1 : Constant  Value=simIn.param.ATC.INPUT_TC  VectorParams1D=off
  Constant2 : Constant  Value=simIn.param.dt  VectorParams1D=off
  Constant3 : Constant  Value=0  VectorParams1D=off  OutDataTypeStr=single
  Data Type Conversion : DataTypeConversion  OutDataTypeStr=single  SaturateOnIntegerOverflow=off  RndMeth=Floor
  Data Type Conversion1 : DataTypeConversion  OutDataTypeStr=single  SaturateOnIntegerOverflow=off  RndMeth=Floor
  MATLAB Function : MATLAB Function  TreatAsAtomicUnit=on
  MATLAB Function1 : MATLAB Function  TreatAsAtomicUnit=on
  Square Root Controller : MATLAB Function  TreatAsAtomicUnit=on
  Square Root Controller1 : Subsystem  TreatAsAtomicUnit=on
  calc p from input_tc : Subsystem
  eulerRollRateTar : Outport
  wires:
  rollAngleErr/1 -> MATLAB Function/1(radIn)
  MATLAB Function/1(radLim) -> Square Root Controller/1(err)
  rollAccelMax/1 -> [accelMax]
  Constant/1 -> Data Type Conversion/1
  Constant1/1 -> calc p from input_tc/1(input_tc)
  calc p from input_tc/1(p) -> Square Root Controller/2(p)
  Square Root Controller/1(correction_rate) -> MATLAB Function1/1(desiredAngVel)
  Constant2/1 -> Data Type Conversion1/1
  [accelMax] -> Square Root Controller/3(second_ord_lim)
  [accelMax] -> MATLAB Function1/3(accelMax)
  MATLAB Function1/1(eulerRateTar) -> eulerRollRateTar/1
  rollRateTarIn/1 -> MATLAB Function1/2(targetAngVel)
  Data Type Conversion/1 -> Square Root Controller/4(dt)
  Data Type Conversion1/1 -> MATLAB Function1/4(dt)
  Constant3/1 -> MATLAB Function1/5(input_tc)
